simulink model "Typ3SimulinkModell"  (R2024a)
settings: Solver=ode23t  StartTime=0.0  StopTime=simTime  MaxStep=1e-7  RelTol=1e-6  EnableMultiTasking=on
values from neighbouring files (symbols this model uses):
  dutyCycleRun = 0.25    [Typ3ModellParameter.m]
  dutyCycleStart = 0    [Typ3ModellParameter.m]
  dutystepTime = 15e-3    (= 0.015)    [Typ3ModellParameter.m]
  fs = 100e3    (= 100000)    [Typ3ModellParameter.m]
  R = 20    [Typ3ModellParameter.m]    (also in Typ3SymbolischeBerechnung_d2.m = 1000; Typ3Uebersetzung.m = 500)
  u1 = 15    [Typ3ModellParameter.m]
  u1ini = 12    [Typ3ModellParameter.m]
  u1stepTime = 35e-3    (= 0.035)    [Typ3ModellParameter.m]
libraries: fl_lib x32, nesl_utility x19, powerlib_extras x4, simulink x2
settings Model: Creator=ich  LastModifiedBy=danie
settings SolverCC: AlgebraicLoopSolver=TrustRegion
settings DataIOCC: LimitDataPoints=on  SaveFormat=Array  SignalLoggingSaveFormat=ModelDataLogs  ReturnWorkspaceOutputs=off
settings OptimizationCC: ExpressionDepthLimit=2147483647  LifeSpan=inf
settings DebuggingCC: UnderspecifiedInitializationDetection=Classic  MergeDetectMultiDrivingBlocksExec=none  SolverPrmCheckMsg=warning  FcnCallInpInsideContextMsg=warning  UnconnectedInputMsg=warning  UnconnectedOutputMsg=warning  UnconnectedLineMsg=warning  StateNameClashWarn=warning  SFUnexpectedBacktrackingDiag=warning  SFNoUnconditionalDefaultTransitionDiag=warning  SFExecutionAtInitializationDiag=none  ArithmeticOperatorsInVariantConditions=warning
settings HardwareCC: ProdBitPerPointer=32  ProdBitPerSizeT=32  ProdBitPerPtrDiffT=32  ProdLargestAtomicFloat=None  ProdIntDivRoundTo=Undefined  ProdEndianess=Unspecified  ProdWordSize=32  ProdHWDeviceType=32-bit Generic
settings ModelReferenceCC: EnableRefExpFcnMdlSchedulingChecks=on  PropagateSignalLabelsOutOfModel=off
settings SFSimCC: SimUseLocalCustomCode=off  CustomCodeUndefinedFunction=UseInterfaceOnly
settings RTWCC: RTWUseLocalCustomCode=off  GPUComputeCapability=3.5  DLArmComputeVersion=19.05
settings CodeAppCC: StateflowObjectComments=on
settings GRTTargetCC: TargetLangStandard=C89/C90 (ANSI)  CombineOutputUpdateFcns=off  GRTInterface=on
settings ConfigComp: CovMetricSettings=dw  CovSaveCumulativeToWorkspaceVar=on  CovSaveSingleToWorkspaceVar=on  CovExternalEMLEnable=off
settings SimscapeCC: SimscapeNormalizeSystem=off

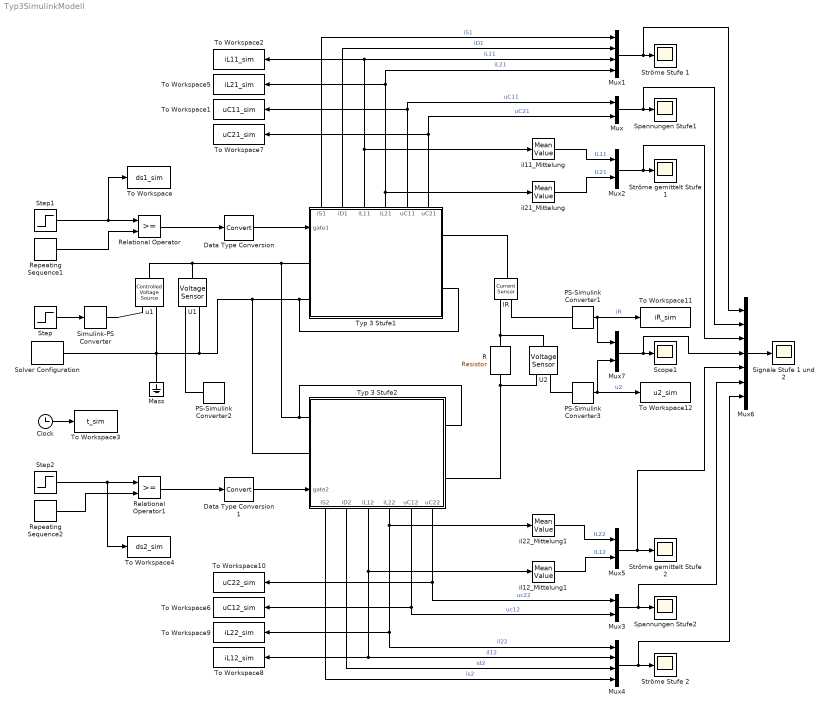
== system Typ3SimulinkModell ==
  Clock : Clock
  Data Type Conversion : DataTypeConversion  SaturateOnIntegerOverflow=off  RndMeth=Floor
  Data Type Conversion1 : DataTypeConversion  SaturateOnIntegerOverflow=off  RndMeth=Floor
  IR : fl_lib/Electrical/Electrical Sensors/Current Sensor
  Mass : fl_lib/Electrical/Electrical Elements/Electrical Reference
  Mux{,2..3,5,7} (5 alike) : Mux  Inputs=2
  Mux1 : Mux
  Mux4 : Mux
  Mux6 : Mux  Inputs=7
  PS-Simulink Converter1 : nesl_utility/PS-Simulink Converter  PhysicalDomain=network_engine_domain  SubClassName=ps_output  LeftPortType=input  RightPortType=output  PseudoPeriodic=off  Frequencies=[]  VectorFormat=1-D array  Unit=1  AffineConversion=off
  PS-Simulink Converter2 : nesl_utility/PS-Simulink Converter  PhysicalDomain=network_engine_domain  SubClassName=ps_output  LeftPortType=input  RightPortType=output  PseudoPeriodic=off  Frequencies=[]  VectorFormat=1-D array  Unit=1  AffineConversion=off
  PS-Simulink Converter3 : nesl_utility/PS-Simulink Converter  PhysicalDomain=network_engine_domain  SubClassName=ps_output  LeftPortType=input  RightPortType=output  PseudoPeriodic=off  Frequencies=[]  VectorFormat=1-D array  Unit=1  AffineConversion=off
  R : fl_lib/Electrical/Electrical Elements/Resistor  R=R Ohm  i_specify=off  i_priority=None  i=0 A  i_nominal_specify=off  i_nominal_value=1  i_nominal_unit=A  v_specify=off  v_priority=None  v=0 V  v_nominal_specify=off  v_nominal_value=1  v_nominal_unit=V
  Relational Operator : RelationalOperator  OutDataTypeStr=boolean  InputSameDT=off
  Relational Operator1 : RelationalOperator  OutDataTypeStr=boolean  InputSameDT=off
  Repeating Sequence1 : simulink/Sources/Repeating Sequence  rep_seq_t=[0 1/(fs)]  rep_seq_y=[0 1]
  Repeating Sequence2 : simulink/Sources/Repeating Sequence  rep_seq_t=[0 1/(fs)]  rep_seq_y=[0 1]
  Scope1 : Scope
  Signale Stufe 1 und 2 : Scope
  Simulink-PS Converter : nesl_utility/Simulink-PS Converter  PhysicalDomain=network_engine_domain  SubClassName=ps_input  LeftPortType=input  RightPortType=output  PseudoPeriodic=off  Frequencies=[]  NoiseDistribution=none  NoiseParameters=[]  Unit=1  AffineConversion=off  FilteringAndDerivatives=zero  SimscapeFilterOrder=1  InputFilterTimeConstant=.001  UdotUserProvided=0
  Solver Configuration : nesl_utility/Solver Configuration  PhysicalDomain=network_engine_domain  SubClassName=solver  LeftPortType=input  RightPortType=generic  Tones=[]  Harmonics=[]  SimulateNoise=off  Profile=off  UseLocalSampling=off  EnableSwitchedLinearOptims=on  FrequencyDomain=off  UseCCode=off  RelTol=0.001  AbsTol=1e-06  MinStep=1e-09  ToWorkspace=off  RevertToSquareIcSolve=off  NumHomotopyIterations=100  PhasorMode=off  PhasorModeNumHarmonics=1  ConsistencySolver=NEWTON_FTOL  IndexReductionMethod=DerivativeReplacement  DoDC=off  ResidualTolerance=1e-9  ConsistencyTolSource=GLOBAL  ConsistencyAbsTol=0.001  ConsistencyRelTol=0.001  ConsistencyTolFactor=0.001  UseLocalSolver=off  LocalSolverChoice=NE_BACKWARD_EULER_ADVANCER  ResolveIndetEquations=on  FunctionEvalNumThread=1  LocalSolverSampleTime=.001  DoFixedCost=off  MaxNonlinIter=3  MaxModeIter=2  ComputeImpulses=off  ImpulseIterations=2  LinearAlgebra=Sparse  LinearAlgebraNumThread=0  EquationFormulation=NE_TIME_EF  DelaysMemoryBudget=1024  AutomaticFiltering=on  FilteringTimeConstant=0.001  PartitionStorageMethod=AS_NEEDED  PartitionMemoryBudget=1024  PartitionMethod=FAST  MultibodyUseLocalSolver=off  MultibodyLocalSolverChoice=ODE1  MultibodyLocalSolverSampleTime=0.001
  Spannungen Stufe1 : Scope
  Spannungen Stufe2 : Scope
  Step : Step  Time=u1stepTime  Before=u1ini  After=u1  SampleTime=0
  Step1 : Step  Time=dutystepTime  Before=dutyCycleStart  After=dutyCycleRun  SampleTime=0
  Step2 : Step  Time=dutystepTime  Before=dutyCycleStart  After=dutyCycleRun  SampleTime=0
  Ströme Stufe 1 : Scope
  Ströme Stufe 2 : Scope
  Ströme gemittelt Stufe 1 : Scope
  Ströme gemittelt Stufe 2 : Scope
  To Workspace : ToWorkspace  VariableName=ds1_sim  SampleTime=-1
  To Workspace1 : ToWorkspace  VariableName=uC11_sim  SampleTime=-1
  To Workspace10 : ToWorkspace  VariableName=uC22_sim  SampleTime=-1
  To Workspace11 : ToWorkspace  VariableName=iR_sim  SampleTime=-1
  To Workspace12 : ToWorkspace  VariableName=u2_sim  SampleTime=-1
  To Workspace2 : ToWorkspace  VariableName=iL11_sim  SampleTime=-1
  To Workspace3 : ToWorkspace  VariableName=t_sim  SampleTime=-1
  To Workspace4 : ToWorkspace  VariableName=ds2_sim  SampleTime=-1
  To Workspace5 : ToWorkspace  VariableName=iL21_sim  SampleTime=-1
  To Workspace6 : ToWorkspace  VariableName=uC12_sim  SampleTime=-1
  To Workspace7 : ToWorkspace  VariableName=uC21_sim  SampleTime=-1
  To Workspace8 : ToWorkspace  VariableName=iL12_sim  SampleTime=-1
  To Workspace9 : ToWorkspace  VariableName=iL22_sim  SampleTime=-1
  Typ 3 Stufe1 : Subsystem
      settings: PortSchema="{\"entries\":[{\"content\":{\"sides\":[{\"content\":{\"connectorIds\":[\"In1\",\"LConn1\",\"LConn2\"]},\"type\":\"ConnectorPlacement.EquallySpacedRectSide\",\"uuid\":\"4689dcfc-a571-4b44-afe3-81c51c9efd0b\"},{\"content\":{\"connectorIds\":[\"RConn1\",\"RConn2\"],\"side\":\"RIGHT\"},\"type\":\"ConnectorPlacement.EquallySpacedRectSide\",\"uuid\":\"2d9a0775-4bf2-455c-8ce1-129bcedaf02a\"},{\"content\":{\"connectorIds\":[\"Out1\",\"Out2\",\"Out3\",\"Out4\",\"Out5\",\"Out6\"],\"side\":\"TOP\"},\"type\":\"ConnectorPlacement.EquallySpacedRectSide\",\"uuid\":\"ff5cf8d4-2a7a-404f-9741-a5db3d17d735\"}]},\"type\":\"ConnectorPlacement.EquallySpacedConnector\",\"uuid\":\"7ae0b5fb-2280-459f-abff-01da95914651\"}],\"packageUris\":[\"http://schema.mathworks.com/mf0/Connector/R2020b\"],\"version\":\"1.0\"}"
  Typ 3 Stufe2 : Subsystem
      settings: PortSchema="{\"entries\":[{\"content\":{\"sides\":[{\"content\":{\"connectorIds\":[\"LConn1\",\"LConn2\",\"In1\"]},\"type\":\"ConnectorPlacement.EquallySpacedRectSide\",\"uuid\":\"4689dcfc-a571-4b44-afe3-81c51c9efd0b\"},{\"content\":{\"connectorIds\":[\"RConn1\",\"RConn2\"],\"side\":\"RIGHT\"},\"type\":\"ConnectorPlacement.EquallySpacedRectSide\",\"uuid\":\"2d9a0775-4bf2-455c-8ce1-129bcedaf02a\"},{\"content\":{\"side\":\"TOP\"},\"type\":\"ConnectorPlacement.EquallySpacedRectSide\",\"uuid\":\"ff5cf8d4-2a7a-404f-9741-a5db3d17d735\"},{\"content\":{\"connectorIds\":[\"Out1\",\"Out2\",\"Out3\",\"Out4\",\"Out5\",\"Out6\"],\"side\":\"BOTTOM\"},\"type\":\"ConnectorPlacement.EquallySpacedRectSide\",\"uuid\":\"6bf6aa49-e12a-46c9-8110-ab80b6ad5f47\"}]},\"type\":\"ConnectorPlacement.EquallySpacedConnector\",\"uuid\":\"7ae0b5fb-2280-459f-abff-01da95914651\"}],\"packageUris\":[\"http://schema.mathworks.com/mf0/Connector/R2020b\"],\"version\":\"1.0\"}"
  U1 : fl_lib/Electrical/Electrical Sensors/Voltage Sensor
  U2 : fl_lib/Electrical/Electrical Sensors/Voltage Sensor
  il11_Mittelung : powerlib_extras/Measurements/Mean Value  Period=1/(50e3)
  il12_Mittelung1 : powerlib_extras/Measurements/Mean Value  Period=1/(50e3)
  il21_Mittelung : powerlib_extras/Measurements/Mean Value  Period=1/(50e3)
  il22_Mittelung1 : powerlib_extras/Measurements/Mean Value  Period=1/(50e3)
  u1 : fl_lib/Electrical/Electrical Sources/Controlled Voltage Source
  wires:
  Step/1 -> Simulink-PS Converter/1
  Step1/1 -> To Workspace/1, Relational Operator/1
  Mux/1 -> Mux6/2, Spannungen Stufe1/1
  Mux1/1 -> Mux6/1, Ströme Stufe 1/1
  Relational Operator/1 -> Data Type Conversion/1
  Clock/1 -> To Workspace3/1
  PS-Simulink Converter3/1 -> Mux7/2, To Workspace12/1  "u2"
  Step2/1 -> Relational Operator1/1, To Workspace4/1
  Repeating Sequence1/1 -> Relational Operator/2
  Data Type Conversion/1 -> Typ 3 Stufe1/1(gate1)
  Typ 3 Stufe1/1(iS1) -> Mux1/1  "iS1"
  Typ 3 Stufe1/2(iD1) -> Mux1/2  "iD1"
  Typ 3 Stufe1/3(iL11) -> Mux1/3, To Workspace2/1, il11_Mittelung/1  "iL11"
  Typ 3 Stufe1/4(iL21) -> il21_Mittelung/1, To Workspace5/1, Mux1/4  "iL21"
  Typ 3 Stufe1/6(uC21) -> Mux/2, To Workspace7/1  "uC21"
  Typ 3 Stufe1/5(uC11) -> Mux/1, To Workspace1/1  "uC11"
  il11_Mittelung/1 -> Mux2/1  "IL11"
  il21_Mittelung/1 -> Mux2/2  "IL21"
  Mux3/1 -> Mux6/6, Spannungen Stufe2/1
  Mux4/1 -> Mux6/7, Ströme Stufe 2/1
  Mux5/1 -> Mux6/5, Ströme gemittelt Stufe 2/1
  il12_Mittelung1/1 -> Mux5/2  "IL12"
  il22_Mittelung1/1 -> Mux5/1  "IL22"
  Typ 3 Stufe2/1(iS2) -> Mux4/4  "is2"
  Typ 3 Stufe2/2(iD2) -> Mux4/3  "id2"
  Typ 3 Stufe2/3(iL12) -> Mux4/2, To Workspace8/1, il12_Mittelung1/1  "il12"
  Typ 3 Stufe2/4(iL22) -> To Workspace9/1, Mux4/1, il22_Mittelung1/1  "il22"
  Typ 3 Stufe2/5(uC12) -> To Workspace6/1, Mux3/2  "uc12"
  Typ 3 Stufe2/6(uC22) -> To Workspace10/1, Mux3/1  "uc22"
  Mux7/1 -> Scope1/1, Mux6/4
  PS-Simulink Converter1/1 -> Mux7/1, To Workspace11/1  "iR"
  Data Type Conversion1/1 -> Typ 3 Stufe2/1(gate2)
  Relational Operator1/1 -> Data Type Conversion1/1
  Repeating Sequence2/1 -> Relational Operator1/2
  Mux2/1 -> Ströme gemittelt Stufe 1/1, Mux6/3
  Mux6/1 -> Signale Stufe 1 und 2/1
  connections:
  Simulink-PS Converter/RConn1 -- u1/RConn1
  R/LConn1 -- Typ 3 Stufe2/RConn2 -- U2/RConn2
  R/RConn1 -- IR/RConn2 -- U2/LConn1
  Typ 3 Stufe1/LConn1 -- Typ 3 Stufe2/RConn1 -- Typ 3 Stufe2/LConn1 -- u1/LConn1 -- U1/LConn1
  u1/RConn2 -- Typ 3 Stufe2/LConn2 -- Typ 3 Stufe1/RConn2 -- Typ 3 Stufe1/LConn2 -- U1/RConn2 -- Mass/LConn1 -- Solver Configuration/RConn1
  U1/RConn1 -- PS-Simulink Converter2/LConn1
  PS-Simulink Converter3/LConn1 -- U2/RConn1
  IR/LConn1 -- Typ 3 Stufe1/RConn1
  PS-Simulink Converter1/LConn1 -- IR/RConn1

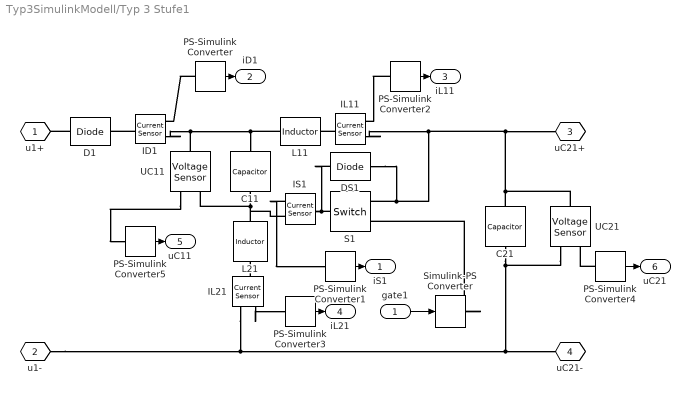
== system Typ3SimulinkModell/Typ 3 Stufe1 ==
  gate1 : Inport
  C11 : fl_lib/Electrical/Electrical Elements/Capacitor  c=C11 F  r=RC11 Ohm  g=0 1/Ohm  i_specify=off  i_priority=None  i=0 A  i_nominal_specify=off  i_nominal_value=1  i_nominal_unit=A  v_specify=off  v_priority=None  v=0 V  v_nominal_specify=off  v_nominal_value=1  v_nominal_unit=V  vc_specify=on  vc_priority=High  vc=0 V  vc_nominal_specify=off  vc_nominal_value=1  vc_nominal_unit=V
  C21 : fl_lib/Electrical/Electrical Elements/Capacitor  c=C21 F  r=RC21 Ohm  g=0 1/Ohm  i_specify=off  i_priority=None  i=0 A  i_nominal_specify=off  i_nominal_value=1  i_nominal_unit=A  v_specify=off  v_priority=None  v=0 V  v_nominal_specify=off  v_nominal_value=1  v_nominal_unit=V  vc_specify=on  vc_priority=High  vc=0 V  vc_nominal_specify=off  vc_nominal_value=1  vc_nominal_unit=V
  D1 : fl_lib/Electrical/Electrical Elements/Diode  Vf=UD1 V  Ron=RD1 Ohm  Goff=1e-9 1/Ohm  i_specify=off  i_priority=None  i=0 A  i_nominal_specify=off  i_nominal_value=1  i_nominal_unit=A  v_specify=off  v_priority=None  v=0 V  v_nominal_specify=off  v_nominal_value=1  v_nominal_unit=V
  DS1 : fl_lib/Electrical/Electrical Elements/Diode  Vf=UDS1 V  Ron=RS1 Ohm  Goff=1e-9 1/Ohm  i_specify=off  i_priority=None  i=0 A  i_nominal_specify=off  i_nominal_value=1  i_nominal_unit=A  v_specify=off  v_priority=None  v=0 V  v_nominal_specify=off  v_nominal_value=1  v_nominal_unit=V
  ID1 : fl_lib/Electrical/Electrical Sensors/Current Sensor
  IL11 : fl_lib/Electrical/Electrical Sensors/Current Sensor
  IL21 : fl_lib/Electrical/Electrical Sensors/Current Sensor
  IS1 : fl_lib/Electrical/Electrical Sensors/Current Sensor
  L11 : fl_lib/Electrical/Electrical Elements/Inductor  l=L11 H  r=RL11 Ohm  g=1e-9 1/Ohm  i_specify=off  i_priority=None  i=0 A  i_nominal_specify=off  i_nominal_value=1  i_nominal_unit=A  v_specify=off  v_priority=None  v=0 V  v_nominal_specify=off  v_nominal_value=1  v_nominal_unit=V  i_L_specify=on  i_L_priority=High  i_L=0 A  i_L_nominal_specify=off  i_L_nominal_value=1  i_L_nominal_unit=A
  L21 : fl_lib/Electrical/Electrical Elements/Inductor  l=L21 H  r=RL21 Ohm  g=1e-9 1/Ohm  i_specify=off  i_priority=None  i=0 A  i_nominal_specify=off  i_nominal_value=1  i_nominal_unit=A  v_specify=off  v_priority=None  v=0 V  v_nominal_specify=off  v_nominal_value=1  v_nominal_unit=V  i_L_specify=on  i_L_priority=High  i_L=0 A  i_L_nominal_specify=off  i_L_nominal_value=1  i_L_nominal_unit=A
  PS-Simulink Converter{,1..5} (6 alike) : nesl_utility/PS-Simulink Converter  PhysicalDomain=network_engine_domain  SubClassName=ps_output  LeftPortType=input  RightPortType=output  PseudoPeriodic=off  Frequencies=[]  VectorFormat=1-D array  Unit=1  AffineConversion=off
  S1 : fl_lib/Electrical/Electrical Elements/Switch  R_closed=RS1 Ohm  G_open=1e-9 1/Ohm  Threshold=0.5  i_specify=off  i_priority=None  i=0 A  i_nominal_specify=off  i_nominal_value=1  i_nominal_unit=A  v_specify=off  v_priority=None  v=0 V  v_nominal_specify=off  v_nominal_value=1  v_nominal_unit=V
  Simulink-PS Converter : nesl_utility/Simulink-PS Converter  PhysicalDomain=network_engine_domain  SubClassName=ps_input  LeftPortType=input  RightPortType=output  PseudoPeriodic=off  Frequencies=[]  NoiseDistribution=none  NoiseParameters=[]  Unit=1  AffineConversion=off  FilteringAndDerivatives=zero  SimscapeFilterOrder=1  InputFilterTimeConstant=.001  UdotUserProvided=0
  UC11 : fl_lib/Electrical/Electrical Sensors/Voltage Sensor
  UC21 : fl_lib/Electrical/Electrical Sensors/Voltage Sensor
  u1+ : PMIOPort  Tag=PMCPort  Side=Left
  u1- : PMIOPort  Tag=PMCPort  Port=2  Side=Left
  uC21+ : PMIOPort  Tag=PMCPort  Port=3  Side=Right
  uC21- : PMIOPort  Tag=PMCPort  Port=4  Side=Right
  iS1 : Outport
  iD1 : Outport  Port=2
  iL11 : Outport  Port=3
  iL21 : Outport  Port=4
  uC11 : Outport  Port=5
  uC21 : Outport  Port=6
  wires:
  PS-Simulink Converter3/1 -> iL21/1
  PS-Simulink Converter/1 -> iD1/1
  gate1/1 -> Simulink-PS Converter/1
  PS-Simulink Converter1/1 -> iS1/1
  PS-Simulink Converter2/1 -> iL11/1
  PS-Simulink Converter4/1 -> uC21/1
  PS-Simulink Converter5/1 -> uC11/1
  connections:
  PS-Simulink Converter/LConn1 -- ID1/RConn1
  IL21/RConn1 -- PS-Simulink Converter3/LConn1
  IS1/RConn1 -- PS-Simulink Converter1/LConn1
  Simulink-PS Converter/RConn1 -- S1/RConn1
  L11/LConn1 -- ID1/RConn2 -- UC11/LConn1 -- C11/LConn1
  u1-/RConn1 -- UC21/RConn2 -- C21/RConn1 -- uC21-/RConn1 -- IL21/RConn2
  IL11/RConn2 -- C21/LConn1 -- UC21/LConn1 -- uC21+/RConn1 -- DS1/RConn1 -- S1/RConn2
  IL11/LConn1 -- L11/RConn1
  PS-Simulink Converter2/LConn1 -- IL11/RConn1
  D1/LConn1 -- u1+/RConn1
  IS1/RConn2 -- UC11/RConn2 -- L21/LConn1 -- C11/RConn1
  S1/LConn1 -- DS1/LConn1 -- IS1/LConn1
  IL21/LConn1 -- L21/RConn1
  ID1/LConn1 -- D1/RConn1
  PS-Simulink Converter4/LConn1 -- UC21/RConn1
  UC11/RConn1 -- PS-Simulink Converter5/LConn1

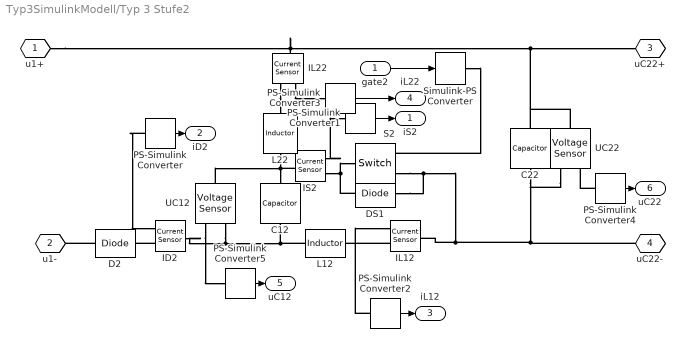
== system Typ3SimulinkModell/Typ 3 Stufe2 ==
  gate2 : Inport
  C12 : fl_lib/Electrical/Electrical Elements/Capacitor  c=C12 F  r=RC12 Ohm  g=0 1/Ohm  i_specify=off  i_priority=None  i=0 A  i_nominal_specify=off  i_nominal_value=1  i_nominal_unit=A  v_specify=off  v_priority=None  v=0 V  v_nominal_specify=off  v_nominal_value=1  v_nominal_unit=V  vc_specify=on  vc_priority=High  vc=0 V  vc_nominal_specify=off  vc_nominal_value=1  vc_nominal_unit=V
  C22 : fl_lib/Electrical/Electrical Elements/Capacitor  c=C22 F  r=RC22 Ohm  g=0 1/Ohm  i_specify=off  i_priority=None  i=0 A  i_nominal_specify=off  i_nominal_value=1  i_nominal_unit=A  v_specify=off  v_priority=None  v=0 V  v_nominal_specify=off  v_nominal_value=1  v_nominal_unit=V  vc_specify=on  vc_priority=High  vc=0 V  vc_nominal_specify=off  vc_nominal_value=1  vc_nominal_unit=V
  D2 : fl_lib/Electrical/Electrical Elements/Diode  Vf=UD2 V  Ron=RD2 Ohm  Goff=1e-9 1/Ohm  i_specify=off  i_priority=None  i=0 A  i_nominal_specify=off  i_nominal_value=1  i_nominal_unit=A  v_specify=off  v_priority=None  v=0 V  v_nominal_specify=off  v_nominal_value=1  v_nominal_unit=V
  DS1 : fl_lib/Electrical/Electrical Elements/Diode  Vf=UDS1 V  Ron=RS1 Ohm  Goff=1e-9 1/Ohm  i_specify=off  i_priority=None  i=0 A  i_nominal_specify=off  i_nominal_value=1  i_nominal_unit=A  v_specify=off  v_priority=None  v=0 V  v_nominal_specify=off  v_nominal_value=1  v_nominal_unit=V
  ID2 : fl_lib/Electrical/Electrical Sensors/Current Sensor
  IL12 : fl_lib/Electrical/Electrical Sensors/Current Sensor
  IL22 : fl_lib/Electrical/Electrical Sensors/Current Sensor
  IS2 : fl_lib/Electrical/Electrical Sensors/Current Sensor
  L12 : fl_lib/Electrical/Electrical Elements/Inductor  l=L12 H  r=RL12 Ohm  g=1e-9 1/Ohm  i_specify=off  i_priority=None  i=0 A  i_nominal_specify=off  i_nominal_value=1  i_nominal_unit=A  v_specify=off  v_priority=None  v=0 V  v_nominal_specify=off  v_nominal_value=1  v_nominal_unit=V  i_L_specify=on  i_L_priority=High  i_L=0 A  i_L_nominal_specify=off  i_L_nominal_value=1  i_L_nominal_unit=A
  L22 : fl_lib/Electrical/Electrical Elements/Inductor  l=L22 H  r=RL22 Ohm  g=1e-9 1/Ohm  i_specify=off  i_priority=None  i=0 A  i_nominal_specify=off  i_nominal_value=1  i_nominal_unit=A  v_specify=off  v_priority=None  v=0 V  v_nominal_specify=off  v_nominal_value=1  v_nominal_unit=V  i_L_specify=on  i_L_priority=High  i_L=0 A  i_L_nominal_specify=off  i_L_nominal_value=1  i_L_nominal_unit=A
  PS-Simulink Converter{,1..5} (6 alike) : nesl_utility/PS-Simulink Converter  PhysicalDomain=network_engine_domain  SubClassName=ps_output  LeftPortType=input  RightPortType=output  PseudoPeriodic=off  Frequencies=[]  VectorFormat=1-D array  Unit=1  AffineConversion=off
  S2 : fl_lib/Electrical/Electrical Elements/Switch  R_closed=RS2 Ohm  G_open=1e-9 1/Ohm  Threshold=0.5  i_specify=off  i_priority=None  i=0 A  i_nominal_specify=off  i_nominal_value=1  i_nominal_unit=A  v_specify=off  v_priority=None  v=0 V  v_nominal_specify=off  v_nominal_value=1  v_nominal_unit=V
  Simulink-PS Converter : nesl_utility/Simulink-PS Converter  PhysicalDomain=network_engine_domain  SubClassName=ps_input  LeftPortType=input  RightPortType=output  PseudoPeriodic=off  Frequencies=[]  NoiseDistribution=none  NoiseParameters=[]  Unit=1  AffineConversion=off  FilteringAndDerivatives=zero  SimscapeFilterOrder=1  InputFilterTimeConstant=.001  UdotUserProvided=0
  UC12 : fl_lib/Electrical/Electrical Sensors/Voltage Sensor
  UC22 : fl_lib/Electrical/Electrical Sensors/Voltage Sensor
  u1+ : PMIOPort  Tag=PMCPort  Side=Left
  u1- : PMIOPort  Tag=PMCPort  Port=2  Side=Left
  uC22+ : PMIOPort  Tag=PMCPort  Port=3  Side=Right
  uC22- : PMIOPort  Tag=PMCPort  Port=4  Side=Right
  iS2 : Outport
  iD2 : Outport  Port=2
  iL12 : Outport  Port=3
  iL22 : Outport  Port=4
  uC12 : Outport  Port=5
  uC22 : Outport  Port=6
  wires:
  PS-Simulink Converter3/1 -> iL22/1
  PS-Simulink Converter/1 -> iD2/1
  gate2/1 -> Simulink-PS Converter/1
  PS-Simulink Converter1/1 -> iS2/1
  PS-Simulink Converter2/1 -> iL12/1
  PS-Simulink Converter4/1 -> uC22/1
  PS-Simulink Converter5/1 -> uC12/1
  connections:
  PS-Simulink Converter/LConn1 -- ID2/RConn1
  IL22/RConn1 -- PS-Simulink Converter3/LConn1
  IS2/RConn1 -- PS-Simulink Converter1/LConn1
  Simulink-PS Converter/RConn1 -- S2/RConn1
  PS-Simulink Converter2/LConn1 -- IL12/RConn1
  PS-Simulink Converter4/LConn1 -- UC22/RConn1
  UC12/RConn1 -- PS-Simulink Converter5/LConn1
  IL12/RConn2 -- L12/LConn1
  L22/RConn1 -- UC12/LConn1 -- IS2/LConn1 -- C12/LConn1
  UC12/RConn2 -- C12/RConn1 -- L12/RConn1 -- ID2/LConn1
  D2/RConn1 -- u1-/RConn1
  u1+/RConn1 -- IL22/LConn1 -- UC22/LConn1 -- C22/LConn1 -- uC22+/RConn1
  S2/RConn2 -- DS1/LConn1 -- UC22/RConn2 -- C22/RConn1 -- uC22-/RConn1 -- IL12/LConn1
  IL22/RConn2 -- L22/LConn1
  ID2/RConn2 -- D2/LConn1
  IS2/RConn2 -- DS1/RConn1 -- S2/LConn1
